simulink model "BESS_2Q_All_Cases_Pro"  (R2024b)
settings: Solver=VariableStepAuto  StartTime=0.0  StopTime=10  RelTol=1e-3
undefined symbols (not defined in the file): Down, Up
libraries: spsSeriesRLCBranchLib x30, spsIGBTDiodeLib x12, spsDCVoltageSourceLib x12, spsVoltageMeasurementLib x12, spsCurrentMeasurementLib x6, eePwmGenerator x2, slpidlib x2, spspowerguiLib x1
settings Model: Creator=jmy  LastModifiedBy=Eng.Abd-Elrhman Saad

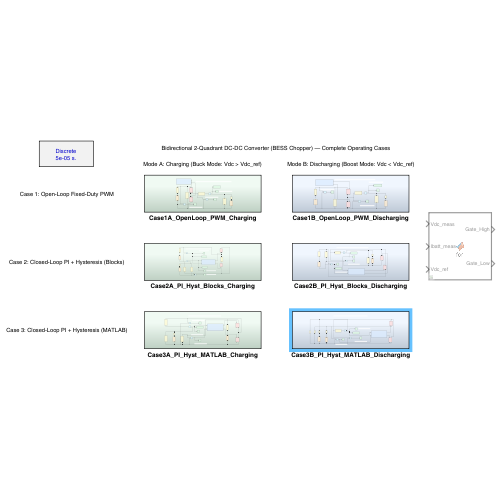
[thumbnail: Simulink's stored preview of the top-level diagram]
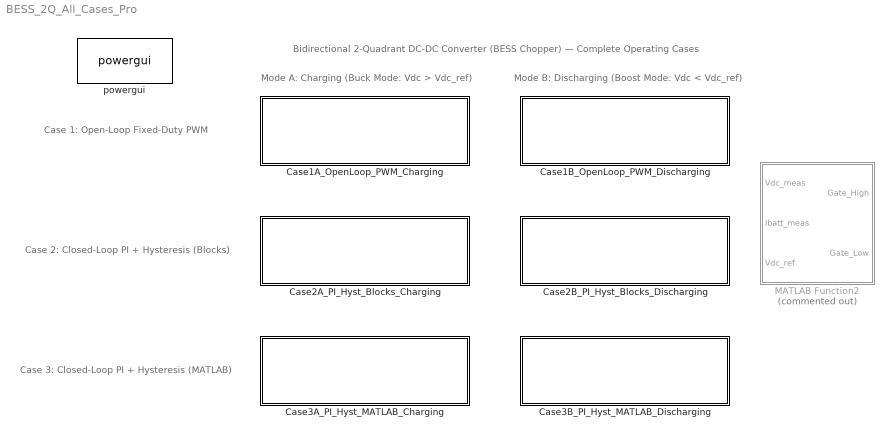
== system BESS_2Q_All_Cases_Pro ==
  note: Bidirectional 2-Quadrant DC-DC Converter (BESS Chopper) — Complete Operating Cases
  note: Mode A: Charging (Buck Mode: Vdc > Vdc_ref)
  note: Mode B: Discharging (Boost Mode: Vdc < Vdc_ref)
  note: Case 1: Open-Loop Fixed-Duty PWM
  note: Case 2: Closed-Loop PI + Hysteresis (Blocks)
  note: Case 3: Closed-Loop PI + Hysteresis (MATLAB)
  Case1A_OpenLoop_PWM_Charging : Subsystem
  Case1B_OpenLoop_PWM_Discharging : Subsystem
  Case2A_PI_Hyst_Blocks_Charging : Subsystem
  Case2B_PI_Hyst_Blocks_Discharging : Subsystem
  Case3A_PI_Hyst_MATLAB_Charging : Subsystem
  Case3B_PI_Hyst_MATLAB_Discharging : Subsystem
  MATLAB Function2 : MATLAB Function  Commented=on  TreatAsAtomicUnit=on
  powergui : spspowerguiLib/powergui  Priority=1  SimulationMode=Discrete  SampleTime=50e-6  frequency=60  Iterations=50  frequencyindice=0  Pbase=100e6  ErrMax=1e-4  UnitsV=kV  UnitsW=MW  buscounter=0  FunctionMessages=off  echomessages=off  EnableUseOfTLC=off  CurrentSourceSwitches=off  DisableSnubberDevices=off  DisableRonSwitches=off  DisableVfSwitches=off  DisplayEquations=off  AutomaticDiscreteSolvers=off  SolverType=Tustin/Backward Euler (TBE)  Interpol=off  ExternalGateDelay=off  methode=off  Ts=100  x0status=blocks  SPID=on  SwTol=0  HookPort=off  NonlinearTolerance=1e-4  nMaxIteration=100  ContinueOnMaxIteration=off  RestoreLinks=warning  ResistiveCurrentMeasurement=off  Frange=[0:2:500]  Ylog=off  Xlog=on  ShowGrid=off  save=off  variable=ZData  structure=0  ZoomFFT=off  StartTime=0.0  cycles=1  DisplayStyle=1  fundamental=60  FreqAxis=off  MaxFrequency=1000  frequencyindicesteady=1  RmsSteady=1  display=off

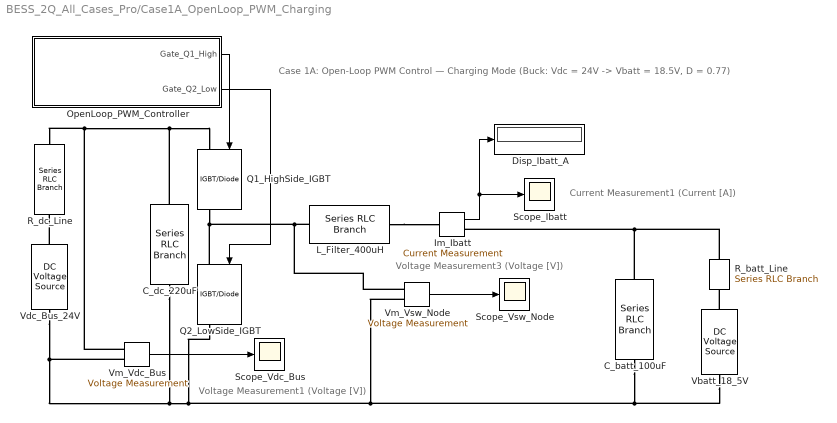
== system BESS_2Q_All_Cases_Pro/Case1A_OpenLoop_PWM_Charging ==
  note: Case 1A: Open-Loop PWM Control — Charging Mode (Buck: Vdc = 24V -> Vbatt = 18.5V, D = 0.77)
  note: Current Measurement1 (Current [A])
  note: Voltage Measurement1 (Voltage [V])
  note: Voltage Measurement3 (Voltage [V])
  C_batt_100uF : spsSeriesRLCBranchLib/Series RLC Branch  LConnTagsString=__new0  RConnTagsString=__new0  BranchType=C  Resistance=1  Inductance=400e-6  SetiL0=off  InitialCurrent=0  Capacitance=100e-6  Setx0=off  InitialVoltage=0  Measurements=None
  C_dc_220uF : spsSeriesRLCBranchLib/Series RLC Branch  LConnTagsString=__new0  RConnTagsString=__new0  BranchType=C  Resistance=1  Inductance=400e-6  SetiL0=off  InitialCurrent=0  Capacitance=220e-6  Setx0=off  InitialVoltage=0  Measurements=None
  Disp_Ibatt_A : Display
  Im_Ibatt : spsCurrentMeasurementLib/Current Measurement  PhasorSimulation=off  OutputType=Complex  PSBequivalent=0
  L_Filter_400uH : spsSeriesRLCBranchLib/Series RLC Branch  LConnTagsString=__new0  RConnTagsString=__new0  BranchType=L  Resistance=1  Inductance=400e-6  SetiL0=off  InitialCurrent=0  Capacitance=1e-6  Setx0=off  InitialVoltage=0  Measurements=None
  OpenLoop_PWM_Controller : Subsystem
  Q1_HighSide_IGBT : spsIGBTDiodeLib/IGBT//Diode  Ron=1e-3  Rs=1e5  Cs=inf  Measurements=on
  Q2_LowSide_IGBT : spsIGBTDiodeLib/IGBT//Diode  Ron=1e-3  Rs=1e5  Cs=inf  Measurements=on
  R_batt_Line : spsSeriesRLCBranchLib/Series RLC Branch  LConnTagsString=__new0  RConnTagsString=__new0  BranchType=R  Resistance=0.0001  Inductance=400e-6  SetiL0=off  InitialCurrent=0  Capacitance=220e-6  Setx0=off  InitialVoltage=0  Measurements=None
  R_dc_Line : spsSeriesRLCBranchLib/Series RLC Branch  LConnTagsString=__new0  RConnTagsString=__new0  BranchType=R  Resistance=0.0001  Inductance=400e-6  SetiL0=off  InitialCurrent=0  Capacitance=220e-6  Setx0=off  InitialVoltage=0  Measurements=None
  Scope_Ibatt : Scope
  Scope_Vdc_Bus : Scope
  Scope_Vsw_Node : Scope
  Vbatt_18_5V : spsDCVoltageSourceLib/DC Voltage Source  Amplitude=18.5  Measurements=None
  Vdc_Bus_24V : spsDCVoltageSourceLib/DC Voltage Source  Amplitude=24  Measurements=None
  Vm_Vdc_Bus : spsVoltageMeasurementLib/Voltage Measurement  PhasorSimulation=off  OutputType=Complex  PSBequivalent=0
  Vm_Vsw_Node : spsVoltageMeasurementLib/Voltage Measurement  PhasorSimulation=off  OutputType=Complex  PSBequivalent=0
  wires:
  Im_Ibatt/1 -> Disp_Ibatt_A/1, Scope_Ibatt/1
  Vm_Vsw_Node/1 -> Scope_Vsw_Node/1
  Vm_Vdc_Bus/1 -> Scope_Vdc_Bus/1
  OpenLoop_PWM_Controller/1(Gate_Q1_High) -> Q1_HighSide_IGBT/1
  OpenLoop_PWM_Controller/2(Gate_Q2_Low) -> Q2_LowSide_IGBT/1
  connections:
  Vbatt_18_5V/RConn1 -- R_batt_Line/RConn1
  Q2_LowSide_IGBT/LConn1 -- Vm_Vsw_Node/LConn1 -- L_Filter_400uH/LConn1 -- Q1_HighSide_IGBT/RConn1
  Vm_Vdc_Bus/LConn1 -- R_dc_Line/LConn1 -- C_dc_220uF/LConn1 -- Q1_HighSide_IGBT/LConn1
  R_batt_Line/LConn1 -- C_batt_100uF/LConn1 -- Im_Ibatt/RConn1
  Vm_Vdc_Bus/LConn2 -- C_dc_220uF/RConn1 -- Vbatt_18_5V/LConn1 -- C_batt_100uF/RConn1 -- Vm_Vsw_Node/LConn2 -- Q2_LowSide_IGBT/RConn1 -- Vdc_Bus_24V/LConn1
  L_Filter_400uH/RConn1 -- Im_Ibatt/LConn1
  Vdc_Bus_24V/RConn1 -- R_dc_Line/RConn1

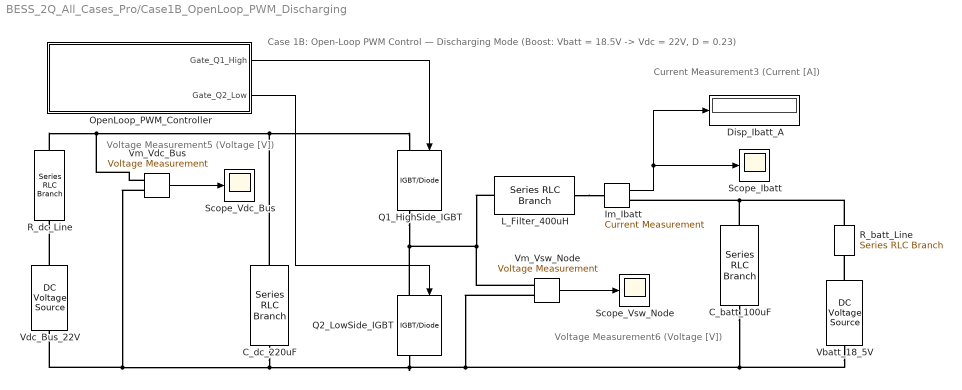
== system BESS_2Q_All_Cases_Pro/Case1B_OpenLoop_PWM_Discharging ==
  note: Case 1B: Open-Loop PWM Control — Discharging Mode (Boost: Vbatt = 18.5V -> Vdc = 22V, D = 0.23)
  note: Current Measurement3 (Current [A])
  note: Voltage Measurement5 (Voltage [V])
  note: Voltage Measurement6 (Voltage [V])
  C_batt_100uF : spsSeriesRLCBranchLib/Series RLC Branch  LConnTagsString=__new0  RConnTagsString=__new0  BranchType=C  Resistance=1  Inductance=400e-6  SetiL0=off  InitialCurrent=0  Capacitance=100e-6  Setx0=off  InitialVoltage=0  Measurements=None
  C_dc_220uF : spsSeriesRLCBranchLib/Series RLC Branch  LConnTagsString=__new0  RConnTagsString=__new0  BranchType=C  Resistance=1  Inductance=400e-6  SetiL0=off  InitialCurrent=0  Capacitance=220e-6  Setx0=off  InitialVoltage=0  Measurements=None
  Disp_Ibatt_A : Display
  Im_Ibatt : spsCurrentMeasurementLib/Current Measurement  PhasorSimulation=off  OutputType=Complex  PSBequivalent=0
  L_Filter_400uH : spsSeriesRLCBranchLib/Series RLC Branch  LConnTagsString=__new0  RConnTagsString=__new0  BranchType=L  Resistance=1  Inductance=400e-6  SetiL0=off  InitialCurrent=0  Capacitance=1e-6  Setx0=off  InitialVoltage=0  Measurements=None
  OpenLoop_PWM_Controller : Subsystem
  Q1_HighSide_IGBT : spsIGBTDiodeLib/IGBT//Diode  Ron=1e-3  Rs=1e5  Cs=inf  Measurements=on
  Q2_LowSide_IGBT : spsIGBTDiodeLib/IGBT//Diode  Ron=1e-3  Rs=1e5  Cs=inf  Measurements=on
  R_batt_Line : spsSeriesRLCBranchLib/Series RLC Branch  LConnTagsString=__new0  RConnTagsString=__new0  BranchType=R  Resistance=0.0001  Inductance=400e-6  SetiL0=off  InitialCurrent=0  Capacitance=220e-6  Setx0=off  InitialVoltage=0  Measurements=None
  R_dc_Line : spsSeriesRLCBranchLib/Series RLC Branch  LConnTagsString=__new0  RConnTagsString=__new0  BranchType=R  Resistance=0.0001  Inductance=400e-6  SetiL0=off  InitialCurrent=0  Capacitance=220e-6  Setx0=off  InitialVoltage=0  Measurements=None
  Scope_Ibatt : Scope
  Scope_Vdc_Bus : Scope
  Scope_Vsw_Node : Scope
  Vbatt_18_5V : spsDCVoltageSourceLib/DC Voltage Source  Amplitude=18.5  Measurements=None
  Vdc_Bus_22V : spsDCVoltageSourceLib/DC Voltage Source  Amplitude=22  Measurements=None
  Vm_Vdc_Bus : spsVoltageMeasurementLib/Voltage Measurement  PhasorSimulation=off  OutputType=Complex  PSBequivalent=0
  Vm_Vsw_Node : spsVoltageMeasurementLib/Voltage Measurement  PhasorSimulation=off  OutputType=Complex  PSBequivalent=0
  wires:
  Vm_Vsw_Node/1 -> Scope_Vsw_Node/1
  Im_Ibatt/1 -> Disp_Ibatt_A/1, Scope_Ibatt/1
  Vm_Vdc_Bus/1 -> Scope_Vdc_Bus/1
  OpenLoop_PWM_Controller/1(Gate_Q1_High) -> Q1_HighSide_IGBT/1
  OpenLoop_PWM_Controller/2(Gate_Q2_Low) -> Q2_LowSide_IGBT/1
  connections:
  Q1_HighSide_IGBT/LConn1 -- Vm_Vdc_Bus/LConn1 -- R_dc_Line/LConn1 -- C_dc_220uF/LConn1
  L_Filter_400uH/RConn1 -- Im_Ibatt/LConn1
  Q2_LowSide_IGBT/RConn1 -- Vdc_Bus_22V/LConn1 -- Vm_Vdc_Bus/LConn2 -- C_dc_220uF/RConn1 -- Vbatt_18_5V/LConn1 -- C_batt_100uF/RConn1 -- Vm_Vsw_Node/LConn2
  Vdc_Bus_22V/RConn1 -- R_dc_Line/RConn1
  Q2_LowSide_IGBT/LConn1 -- Q1_HighSide_IGBT/RConn1 -- L_Filter_400uH/LConn1 -- Vm_Vsw_Node/LConn1
  Vbatt_18_5V/RConn1 -- R_batt_Line/RConn1
  R_batt_Line/LConn1 -- C_batt_100uF/LConn1 -- Im_Ibatt/RConn1

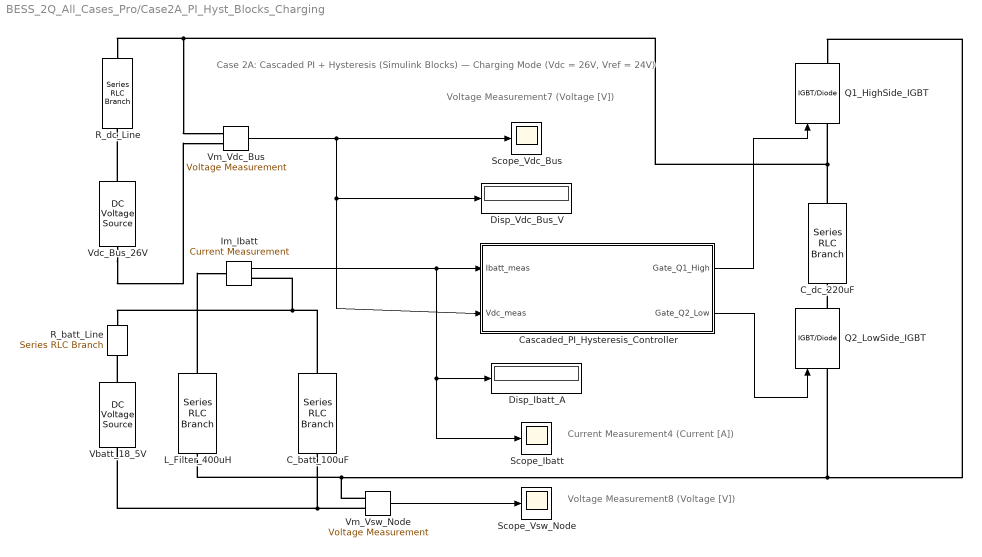
== system BESS_2Q_All_Cases_Pro/Case2A_PI_Hyst_Blocks_Charging ==
  note: Case 2A: Cascaded PI + Hysteresis (Simulink Blocks) — Charging Mode (Vdc = 26V, Vref = 24V)
  note: Current Measurement4 (Current [A])
  note: Voltage Measurement7 (Voltage [V])
  note: Voltage Measurement8 (Voltage [V])
  C_batt_100uF : spsSeriesRLCBranchLib/Series RLC Branch  LConnTagsString=__new0  RConnTagsString=__new0  BranchType=C  Resistance=1  Inductance=400e-6  SetiL0=off  InitialCurrent=0  Capacitance=100e-6  Setx0=off  InitialVoltage=0  Measurements=None
  C_dc_220uF : spsSeriesRLCBranchLib/Series RLC Branch  LConnTagsString=__new0  RConnTagsString=__new0  BranchType=C  Resistance=1  Inductance=400e-6  SetiL0=off  InitialCurrent=0  Capacitance=220e-6  Setx0=off  InitialVoltage=0  Measurements=None
  Cascaded_PI_Hysteresis_Controller : Subsystem
  Disp_Ibatt_A : Display
  Disp_Vdc_Bus_V : Display
  Im_Ibatt : spsCurrentMeasurementLib/Current Measurement  PhasorSimulation=off  OutputType=Complex  PSBequivalent=0
  L_Filter_400uH : spsSeriesRLCBranchLib/Series RLC Branch  LConnTagsString=__new0  RConnTagsString=__new0  BranchType=L  Resistance=1  Inductance=400e-6  SetiL0=off  InitialCurrent=0  Capacitance=1e-6  Setx0=off  InitialVoltage=0  Measurements=None
  Q1_HighSide_IGBT : spsIGBTDiodeLib/IGBT//Diode  Ron=1e-3  Rs=1e5  Cs=inf  Measurements=on
  Q2_LowSide_IGBT : spsIGBTDiodeLib/IGBT//Diode  Ron=1e-3  Rs=1e5  Cs=inf  Measurements=on
  R_batt_Line : spsSeriesRLCBranchLib/Series RLC Branch  LConnTagsString=__new0  RConnTagsString=__new0  BranchType=R  Resistance=0.0001  Inductance=400e-6  SetiL0=off  InitialCurrent=0  Capacitance=220e-6  Setx0=off  InitialVoltage=0  Measurements=None
  R_dc_Line : spsSeriesRLCBranchLib/Series RLC Branch  LConnTagsString=__new0  RConnTagsString=__new0  BranchType=R  Resistance=0.0001  Inductance=400e-6  SetiL0=off  InitialCurrent=0  Capacitance=220e-6  Setx0=off  InitialVoltage=0  Measurements=None
  Scope_Ibatt : Scope
  Scope_Vdc_Bus : Scope
  Scope_Vsw_Node : Scope
  Vbatt_18_5V : spsDCVoltageSourceLib/DC Voltage Source  Amplitude=18.5  Measurements=None
  Vdc_Bus_26V : spsDCVoltageSourceLib/DC Voltage Source  Amplitude=26  Measurements=None
  Vm_Vdc_Bus : spsVoltageMeasurementLib/Voltage Measurement  PhasorSimulation=off  OutputType=Complex  PSBequivalent=0
  Vm_Vsw_Node : spsVoltageMeasurementLib/Voltage Measurement  PhasorSimulation=off  OutputType=Complex  PSBequivalent=0
  wires:
  Vm_Vsw_Node/1 -> Scope_Vsw_Node/1
  Vm_Vdc_Bus/1 -> Disp_Vdc_Bus_V/1, Cascaded_PI_Hysteresis_Controller/2(Vdc_meas), Scope_Vdc_Bus/1
  Im_Ibatt/1 -> Disp_Ibatt_A/1, Scope_Ibatt/1, Cascaded_PI_Hysteresis_Controller/1(Ibatt_meas)
  Cascaded_PI_Hysteresis_Controller/1(Gate_Q1_High) -> Q1_HighSide_IGBT/1
  Cascaded_PI_Hysteresis_Controller/2(Gate_Q2_Low) -> Q2_LowSide_IGBT/1
  connections:
  Vm_Vsw_Node/LConn2 -- Vbatt_18_5V/LConn1 -- C_batt_100uF/RConn1
  Vm_Vsw_Node/LConn1 -- Q2_LowSide_IGBT/LConn1 -- Q1_HighSide_IGBT/RConn1 -- L_Filter_400uH/LConn1
  Vdc_Bus_26V/RConn1 -- R_dc_Line/RConn1
  Vdc_Bus_26V/LConn1 -- Vm_Vdc_Bus/LConn2
  L_Filter_400uH/RConn1 -- Im_Ibatt/LConn1
  Vbatt_18_5V/RConn1 -- R_batt_Line/RConn1
  C_batt_100uF/LConn1 -- Im_Ibatt/RConn1 -- R_batt_Line/LConn1
  Q2_LowSide_IGBT/RConn1 -- C_dc_220uF/RConn1
  C_dc_220uF/LConn1 -- Q1_HighSide_IGBT/LConn1 -- R_dc_Line/LConn1 -- Vm_Vdc_Bus/LConn1

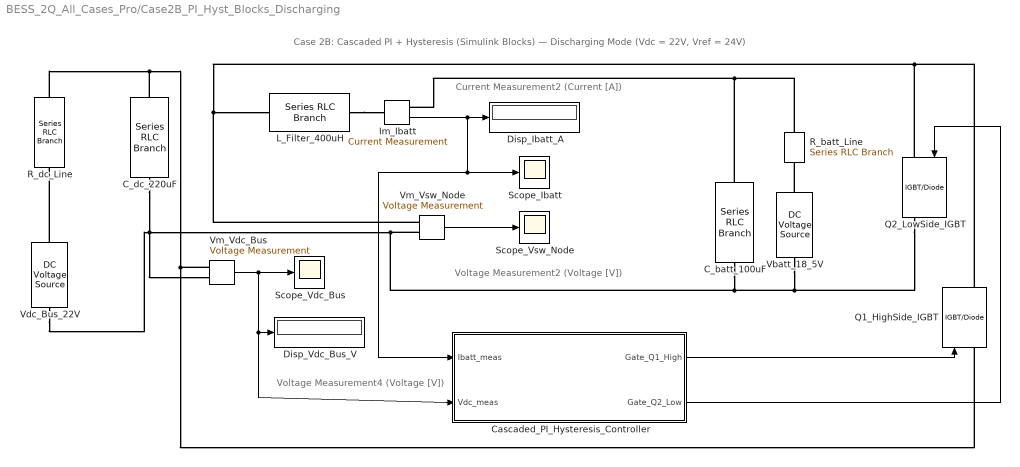
== system BESS_2Q_All_Cases_Pro/Case2B_PI_Hyst_Blocks_Discharging ==
  note: Case 2B: Cascaded PI + Hysteresis (Simulink Blocks) — Discharging Mode (Vdc = 22V, Vref = 24V)
  note: Current Measurement2 (Current [A])
  note: Voltage Measurement2 (Voltage [V])
  note: Voltage Measurement4 (Voltage [V])
  C_batt_100uF : spsSeriesRLCBranchLib/Series RLC Branch  LConnTagsString=__new0  RConnTagsString=__new0  BranchType=C  Resistance=1  Inductance=400e-6  SetiL0=off  InitialCurrent=0  Capacitance=100e-6  Setx0=off  InitialVoltage=0  Measurements=None
  C_dc_220uF : spsSeriesRLCBranchLib/Series RLC Branch  LConnTagsString=__new0  RConnTagsString=__new0  BranchType=C  Resistance=1  Inductance=400e-6  SetiL0=off  InitialCurrent=0  Capacitance=220e-6  Setx0=off  InitialVoltage=0  Measurements=None
  Cascaded_PI_Hysteresis_Controller : Subsystem
  Disp_Ibatt_A : Display
  Disp_Vdc_Bus_V : Display
  Im_Ibatt : spsCurrentMeasurementLib/Current Measurement  PhasorSimulation=off  OutputType=Complex  PSBequivalent=0
  L_Filter_400uH : spsSeriesRLCBranchLib/Series RLC Branch  LConnTagsString=__new0  RConnTagsString=__new0  BranchType=L  Resistance=1  Inductance=400e-6  SetiL0=off  InitialCurrent=0  Capacitance=1e-6  Setx0=off  InitialVoltage=0  Measurements=None
  Q1_HighSide_IGBT : spsIGBTDiodeLib/IGBT//Diode  Ron=1e-3  Rs=1e5  Cs=inf  Measurements=on
  Q2_LowSide_IGBT : spsIGBTDiodeLib/IGBT//Diode  Ron=1e-3  Rs=1e5  Cs=inf  Measurements=on
  R_batt_Line : spsSeriesRLCBranchLib/Series RLC Branch  LConnTagsString=__new0  RConnTagsString=__new0  BranchType=R  Resistance=0.0001  Inductance=400e-6  SetiL0=off  InitialCurrent=0  Capacitance=220e-6  Setx0=off  InitialVoltage=0  Measurements=None
  R_dc_Line : spsSeriesRLCBranchLib/Series RLC Branch  LConnTagsString=__new0  RConnTagsString=__new0  BranchType=R  Resistance=0.0001  Inductance=400e-6  SetiL0=off  InitialCurrent=0  Capacitance=220e-6  Setx0=off  InitialVoltage=0  Measurements=None
  Scope_Ibatt : Scope
  Scope_Vdc_Bus : Scope
  Scope_Vsw_Node : Scope
  Vbatt_18_5V : spsDCVoltageSourceLib/DC Voltage Source  Amplitude=18.5  Measurements=None
  Vdc_Bus_22V : spsDCVoltageSourceLib/DC Voltage Source  Amplitude=22  Measurements=None
  Vm_Vdc_Bus : spsVoltageMeasurementLib/Voltage Measurement  PhasorSimulation=off  OutputType=Complex  PSBequivalent=0
  Vm_Vsw_Node : spsVoltageMeasurementLib/Voltage Measurement  PhasorSimulation=off  OutputType=Complex  PSBequivalent=0
  wires:
  Vm_Vdc_Bus/1 -> Cascaded_PI_Hysteresis_Controller/2(Vdc_meas), Disp_Vdc_Bus_V/1, Scope_Vdc_Bus/1
  Im_Ibatt/1 -> Disp_Ibatt_A/1, Scope_Ibatt/1, Cascaded_PI_Hysteresis_Controller/1(Ibatt_meas)
  Vm_Vsw_Node/1 -> Scope_Vsw_Node/1
  Cascaded_PI_Hysteresis_Controller/1(Gate_Q1_High) -> Q1_HighSide_IGBT/1
  Cascaded_PI_Hysteresis_Controller/2(Gate_Q2_Low) -> Q2_LowSide_IGBT/1
  connections:
  Vdc_Bus_22V/RConn1 -- R_dc_Line/RConn1
  Q2_LowSide_IGBT/RConn1 -- Vbatt_18_5V/LConn1 -- C_batt_100uF/RConn1 -- Vdc_Bus_22V/LConn1 -- Vm_Vdc_Bus/LConn2 -- C_dc_220uF/RConn1 -- Vm_Vsw_Node/LConn2
  Vbatt_18_5V/RConn1 -- R_batt_Line/RConn1
  R_batt_Line/LConn1 -- C_batt_100uF/LConn1 -- Im_Ibatt/RConn1
  Q2_LowSide_IGBT/LConn1 -- Q1_HighSide_IGBT/RConn1 -- Vm_Vsw_Node/LConn1 -- L_Filter_400uH/LConn1
  R_dc_Line/LConn1 -- Q1_HighSide_IGBT/LConn1 -- Vm_Vdc_Bus/LConn1 -- C_dc_220uF/LConn1
  L_Filter_400uH/RConn1 -- Im_Ibatt/LConn1

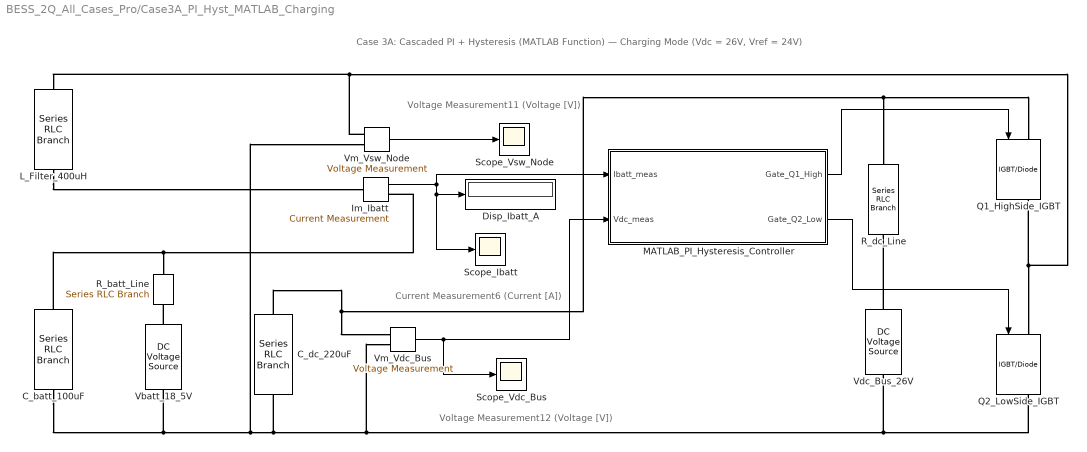
== system BESS_2Q_All_Cases_Pro/Case3A_PI_Hyst_MATLAB_Charging ==
  note: Case 3A: Cascaded PI + Hysteresis (MATLAB Function) — Charging Mode (Vdc = 26V, Vref = 24V)
  note: Current Measurement6 (Current [A])
  note: Voltage Measurement12 (Voltage [V])
  note: Voltage Measurement11 (Voltage [V])
  C_batt_100uF : spsSeriesRLCBranchLib/Series RLC Branch  LConnTagsString=__new0  RConnTagsString=__new0  BranchType=C  Resistance=1  Inductance=400e-6  SetiL0=off  InitialCurrent=0  Capacitance=100e-6  Setx0=off  InitialVoltage=0  Measurements=None
  C_dc_220uF : spsSeriesRLCBranchLib/Series RLC Branch  LConnTagsString=__new0  RConnTagsString=__new0  BranchType=C  Resistance=1  Inductance=400e-6  SetiL0=off  InitialCurrent=0  Capacitance=220e-6  Setx0=off  InitialVoltage=0  Measurements=None
  Disp_Ibatt_A : Display
  Im_Ibatt : spsCurrentMeasurementLib/Current Measurement  PhasorSimulation=off  OutputType=Complex  PSBequivalent=0
  L_Filter_400uH : spsSeriesRLCBranchLib/Series RLC Branch  LConnTagsString=__new0  RConnTagsString=__new0  BranchType=L  Resistance=1  Inductance=400e-6  SetiL0=off  InitialCurrent=0  Capacitance=1e-6  Setx0=off  InitialVoltage=0  Measurements=None
  MATLAB_PI_Hysteresis_Controller : Subsystem
  Q1_HighSide_IGBT : spsIGBTDiodeLib/IGBT//Diode  Ron=1e-3  Rs=1e5  Cs=inf  Measurements=on
  Q2_LowSide_IGBT : spsIGBTDiodeLib/IGBT//Diode  Ron=1e-3  Rs=1e5  Cs=inf  Measurements=on
  R_batt_Line : spsSeriesRLCBranchLib/Series RLC Branch  LConnTagsString=__new0  RConnTagsString=__new0  BranchType=R  Resistance=0.0001  Inductance=400e-6  SetiL0=off  InitialCurrent=0  Capacitance=220e-6  Setx0=off  InitialVoltage=0  Measurements=None
  R_dc_Line : spsSeriesRLCBranchLib/Series RLC Branch  LConnTagsString=__new0  RConnTagsString=__new0  BranchType=R  Resistance=0.0001  Inductance=400e-6  SetiL0=off  InitialCurrent=0  Capacitance=220e-6  Setx0=off  InitialVoltage=0  Measurements=None
  Scope_Ibatt : Scope
  Scope_Vdc_Bus : Scope
  Scope_Vsw_Node : Scope
  Vbatt_18_5V : spsDCVoltageSourceLib/DC Voltage Source  Amplitude=18.5  Measurements=None
  Vdc_Bus_26V : spsDCVoltageSourceLib/DC Voltage Source  Amplitude=26  Measurements=None
  Vm_Vdc_Bus : spsVoltageMeasurementLib/Voltage Measurement  PhasorSimulation=off  OutputType=Complex  PSBequivalent=0
  Vm_Vsw_Node : spsVoltageMeasurementLib/Voltage Measurement  PhasorSimulation=off  OutputType=Complex  PSBequivalent=0
  wires:
  Vm_Vsw_Node/1 -> Scope_Vsw_Node/1
  Vm_Vdc_Bus/1 -> MATLAB_PI_Hysteresis_Controller/2(Vdc_meas), Scope_Vdc_Bus/1
  Im_Ibatt/1 -> Scope_Ibatt/1, Disp_Ibatt_A/1, MATLAB_PI_Hysteresis_Controller/1(Ibatt_meas)
  MATLAB_PI_Hysteresis_Controller/1(Gate_Q1_High) -> Q1_HighSide_IGBT/1
  MATLAB_PI_Hysteresis_Controller/2(Gate_Q2_Low) -> Q2_LowSide_IGBT/1
  connections:
  Vdc_Bus_26V/RConn1 -- R_dc_Line/RConn1
  C_batt_100uF/RConn1 -- Vbatt_18_5V/LConn1 -- C_dc_220uF/RConn1 -- Vm_Vdc_Bus/LConn2 -- Vdc_Bus_26V/LConn1 -- Q2_LowSide_IGBT/RConn1 -- Vm_Vsw_Node/LConn2
  C_batt_100uF/LConn1 -- R_batt_Line/LConn1 -- Im_Ibatt/RConn1
  Vm_Vsw_Node/LConn1 -- L_Filter_400uH/LConn1 -- Q2_LowSide_IGBT/LConn1 -- Q1_HighSide_IGBT/RConn1
  C_dc_220uF/LConn1 -- R_dc_Line/LConn1 -- Q1_HighSide_IGBT/LConn1 -- Vm_Vdc_Bus/LConn1
  Vbatt_18_5V/RConn1 -- R_batt_Line/RConn1
  L_Filter_400uH/RConn1 -- Im_Ibatt/LConn1

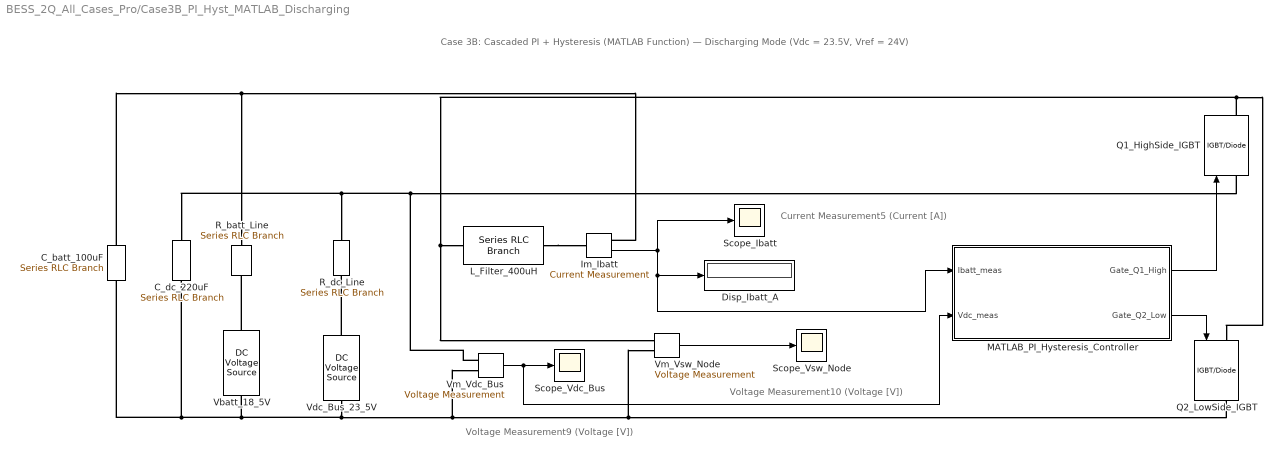
== system BESS_2Q_All_Cases_Pro/Case3B_PI_Hyst_MATLAB_Discharging ==
  note: Case 3B: Cascaded PI + Hysteresis (MATLAB Function) — Discharging Mode (Vdc = 23.5V, Vref = 24V)
  note: Current Measurement5 (Current [A])
  note: Voltage Measurement9 (Voltage [V])
  note: Voltage Measurement10 (Voltage [V])
  C_batt_100uF : spsSeriesRLCBranchLib/Series RLC Branch  LConnTagsString=__new0  RConnTagsString=__new0  BranchType=C  Resistance=1  Inductance=400e-6  SetiL0=off  InitialCurrent=0  Capacitance=100e-6  Setx0=off  InitialVoltage=0  Measurements=None
  C_dc_220uF : spsSeriesRLCBranchLib/Series RLC Branch  LConnTagsString=__new0  RConnTagsString=__new0  BranchType=C  Resistance=1  Inductance=400e-6  SetiL0=off  InitialCurrent=0  Capacitance=220e-6  Setx0=off  InitialVoltage=0  Measurements=None
  Disp_Ibatt_A : Display
  Im_Ibatt : spsCurrentMeasurementLib/Current Measurement  PhasorSimulation=off  OutputType=Complex  PSBequivalent=0
  L_Filter_400uH : spsSeriesRLCBranchLib/Series RLC Branch  LConnTagsString=__new0  RConnTagsString=__new0  BranchType=L  Resistance=1  Inductance=400e-6  SetiL0=off  InitialCurrent=0  Capacitance=1e-6  Setx0=off  InitialVoltage=0  Measurements=None
  MATLAB_PI_Hysteresis_Controller : Subsystem
  Q1_HighSide_IGBT : spsIGBTDiodeLib/IGBT//Diode  Ron=1e-3  Rs=1e5  Cs=inf  Measurements=on
  Q2_LowSide_IGBT : spsIGBTDiodeLib/IGBT//Diode  Ron=1e-3  Rs=1e5  Cs=inf  Measurements=on
  R_batt_Line : spsSeriesRLCBranchLib/Series RLC Branch  LConnTagsString=__new0  RConnTagsString=__new0  BranchType=R  Resistance=0.0001  Inductance=400e-6  SetiL0=off  InitialCurrent=0  Capacitance=220e-6  Setx0=off  InitialVoltage=0  Measurements=None
  R_dc_Line : spsSeriesRLCBranchLib/Series RLC Branch  LConnTagsString=__new0  RConnTagsString=__new0  BranchType=R  Resistance=0.0001  Inductance=400e-6  SetiL0=off  InitialCurrent=0  Capacitance=220e-6  Setx0=off  InitialVoltage=0  Measurements=None
  Scope_Ibatt : Scope
  Scope_Vdc_Bus : Scope
  Scope_Vsw_Node : Scope
  Vbatt_18_5V : spsDCVoltageSourceLib/DC Voltage Source  Amplitude=18.5  Measurements=None
  Vdc_Bus_23_5V : spsDCVoltageSourceLib/DC Voltage Source  Amplitude=23.5  Measurements=None
  Vm_Vdc_Bus : spsVoltageMeasurementLib/Voltage Measurement  PhasorSimulation=off  OutputType=Complex  PSBequivalent=0
  Vm_Vsw_Node : spsVoltageMeasurementLib/Voltage Measurement  PhasorSimulation=off  OutputType=Complex  PSBequivalent=0
  wires:
  Vm_Vdc_Bus/1 -> MATLAB_PI_Hysteresis_Controller/2(Vdc_meas), Scope_Vdc_Bus/1
  Vm_Vsw_Node/1 -> Scope_Vsw_Node/1
  Im_Ibatt/1 -> MATLAB_PI_Hysteresis_Controller/1(Ibatt_meas), Disp_Ibatt_A/1, Scope_Ibatt/1
  MATLAB_PI_Hysteresis_Controller/1(Gate_Q1_High) -> Q1_HighSide_IGBT/1
  MATLAB_PI_Hysteresis_Controller/2(Gate_Q2_Low) -> Q2_LowSide_IGBT/1
  connections:
  Vdc_Bus_23_5V/LConn1 -- C_batt_100uF/RConn1 -- C_dc_220uF/RConn1 -- Vbatt_18_5V/LConn1 -- Vm_Vdc_Bus/LConn2 -- Q2_LowSide_IGBT/RConn1 -- Vm_Vsw_Node/LConn2
  Vdc_Bus_23_5V/RConn1 -- R_dc_Line/RConn1
  Q1_HighSide_IGBT/RConn1 -- Q2_LowSide_IGBT/LConn1 -- L_Filter_400uH/LConn1 -- Vm_Vsw_Node/LConn1
  Vm_Vdc_Bus/LConn1 -- R_dc_Line/LConn1 -- C_dc_220uF/LConn1 -- Q1_HighSide_IGBT/LConn1
  C_batt_100uF/LConn1 -- Im_Ibatt/RConn1 -- R_batt_Line/LConn1
  Vbatt_18_5V/RConn1 -- R_batt_Line/RConn1
  L_Filter_400uH/RConn1 -- Im_Ibatt/LConn1

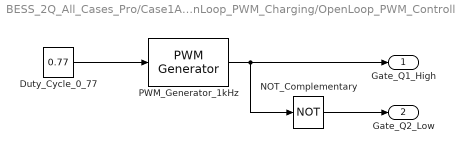
== system BESS_2Q_All_Cases_Pro/Case1A_OpenLoop_PWM_Charging/OpenLoop_PWM_Controller ==
  Duty_Cycle_0_77 : Constant  Value=0.77
  NOT_Complementary : Logic  Operator=NOT  IconShape=distinctive  AllPortsSameDT=off  OutDataTypeStr=boolean
  PWM_Generator_1kHz : eePwmGenerator/PWM Generator  CarrCount=Up-Down  Tper=0.001  Tdelay=0  Ts=5e-5
  Gate_Q1_High : Outport
  Gate_Q2_Low : Outport  Port=2
  wires:
  PWM_Generator_1kHz/1 -> Gate_Q1_High/1, NOT_Complementary/1
  NOT_Complementary/1 -> Gate_Q2_Low/1
  Duty_Cycle_0_77/1 -> PWM_Generator_1kHz/1

== system BESS_2Q_All_Cases_Pro/Case1B_OpenLoop_PWM_Discharging/OpenLoop_PWM_Controller ==
  Duty_Cycle_0_23 : Constant  Value=0.23
  NOT_Complementary : Logic  Operator=NOT  IconShape=distinctive  AllPortsSameDT=off  OutDataTypeStr=boolean
  PWM_Generator_1kHz : eePwmGenerator/PWM Generator  CarrCount=Up-Down  Tper=0.001  Tdelay=0  Ts=5e-5
  Gate_Q1_High : Outport
  Gate_Q2_Low : Outport  Port=2
  wires:
  PWM_Generator_1kHz/1 -> NOT_Complementary/1, Gate_Q2_Low/1
  Duty_Cycle_0_23/1 -> PWM_Generator_1kHz/1
  NOT_Complementary/1 -> Gate_Q1_High/1

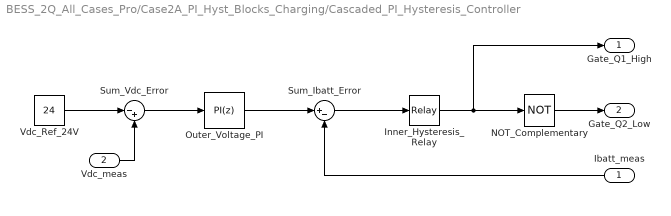
== system BESS_2Q_All_Cases_Pro/Case2A_PI_Hyst_Blocks_Charging/Cascaded_PI_Hysteresis_Controller ==
  Ibatt_meas : Inport
  Vdc_meas : Inport  Port=2
  Inner_Hysteresis_Relay : Relay  OnSwitchValue=0.5  OffSwitchValue=-0.5
  NOT_Complementary : Logic  Operator=NOT  IconShape=distinctive  AllPortsSameDT=off  OutDataTypeStr=boolean
  Outer_Voltage_PI : slpidlib/PID Controller  Controller=PI  Form=Parallel  TimeDomain=Discrete-time  UseExternalTs=off  SampleTime=-1  IntegratorMethod=Forward Euler  FilterMethod=Forward Euler  ControllerParametersSource=internal  P=0.1  I=10  UseKiTs=off  D=0  UseExternalDerivativeSource=off  N=100  UseFilter=on  TunerSelectOption=Transfer Function Based (PID Tuner App)  InitialConditionSource=internal  InitialConditionForIntegrator=0  InitialConditionForFilter=0  DifferentiatorICPrevScaledInput=0  ExternalReset=none  TrackingMode=off  Kt=1  LimitOutput=on  SatLimitsSource=internal  UpperSaturationLimit=3.1  LowerSaturationLimit=-10  LinearizeAsGain=off  AntiWindupMode=none  Kb=1  LimitIntegrator=off  UpperIntegratorSaturationLimit=inf  LowerIntegratorSaturationLimit=-inf  POutMin=[]  POutMax=[]  IOutMin=[]  IOutMax=[]  DOutMin=[]  DOutMax=[]  NOutMin=[]  NOutMax=[]  SumOutMin=[]  SumOutMax=[]  SaturationOutMin=[]  SaturationOutMax=[]  PParamMin=[]  PParamMax=[]  IParamMin=[]  IParamMax=[]  DParamMin=[]  DParamMax=[]  NParamMin=[]  NParamMax=[]  KbParamMin=[]  KbParamMax=[]  KtParamMin=[]  KtParamMax=[]  KbOutMin=[]  KbOutMax=[]  KtOutMin=[]  KtOutMax=[]  IntegratorOutMin=[]  IntegratorOutMax=[]  FilterOutMin=[]  FilterOutMax=[]  SumI1OutMin=[]  SumI1OutMax=[]  SumI2OutMin=[]  SumI2OutMax=[]  SumI3OutMin=[]  SumI3OutMax=[]  SumI4OutMin=[]  SumI4OutMax=[]  SumDOutMin=[]  SumDOutMax=[]  DifferentiatorOutMin=[]  DifferentiatorOutMax=[]  FilterDiffOutCoefMin=[]  FilterDiffOutCoefMax=[]  ReciprocalOutMin=[]  ReciprocalOutMax=[]  SumDenOutMin=[]  SumDenOutMax=[]  SumNumOutMin=[]  SumNumOutMax=[]  DivideOutMin=[]  DivideOutMax=[]  UdiffTsProdOutMin=[]  UdiffTsProdOutMax=[]  NTsProdOutMin=[]  NTsProdOutMax=[]  UintegralTsProdOutMin=[]  UintegralTsProdOutMax=[]  UngainTsProdOutMin=[]  UngainTsProdOutMax=[]  ClampingZeroOutDataTypeStr=Inherit: Inherit via back propagation  ClampingZeroOutMin=[]  ClampingZeroOutMax=[]  FilterDenConstantOutDataTypeStr=Inherit: Inherit via back propagation  FilterDenConstantOutMin=[]  FilterDenConstantOutMax=[]  PCopyOutDataTypeStr=Inherit: Inherit via back propagation  PCopyOutMin=[]  PCopyOutMax=[]  NCopyOutDataTypeStr=Inherit: Inherit via back propagation  NCopyOutMin=[]  NCopyOutMax=[]  IntegratorContinuousStateAttributes=''  IntegratorStateMustResolveToSignalObject=off  IntegratorRTWStateStorageClass=Auto  FilterContinuousStateAttributes=''  FilterStateMustResolveToSignalObject=off  FilterRTWStateStorageClass=Auto  ParallelPVariant=InternalParameters  IdealPVariant=Disabled  IVariant=InternalParameters  DVariant=Disabled  IntegratorVariant=Discrete  SatVariant=Enabled  AWVariant=Passthrough  PCopyVariant=Disabled  TRVariant=Disabled  FdbkBlocksVariant=Forward  IdealPFdbkVariant=Disabled  SatFdbkVariant=Disabled  DerivativeFilterVariant=Disabled  NVariant=Disabled  NCopyVariant=Disabled_SignalSpec  FilterICVariant=Disabled  IntegratorICVariant=InternalICs  ExternalResetVariant=Disabled  TRSumVariant=Passthrough  SumFdbkVariant=Disabled  SumVariant=Sum_PI  TsampFilterVariant=InternalTs  TsampNgainVariant=Passthrough  TsampIntegralVariant=Disabled_SignalSpec  ExternalSaturationOutDataTypeStr=Inherit: Same as second input  DerivativeSourceVariant=Disabled  PreIntVariant=InternalPreInt
  Sum_Ibatt_Error : Sum  Inputs=|+-
  Sum_Vdc_Error : Sum  Inputs=|-+
  Vdc_Ref_24V : Constant  Value=24
  Gate_Q1_High : Outport
  Gate_Q2_Low : Outport  Port=2
  wires:
  Inner_Hysteresis_Relay/1 -> Gate_Q1_High/1, NOT_Complementary/1
  Sum_Vdc_Error/1 -> Outer_Voltage_PI/1
  Outer_Voltage_PI/1 -> Sum_Ibatt_Error/1
  Sum_Ibatt_Error/1 -> Inner_Hysteresis_Relay/1
  NOT_Complementary/1 -> Gate_Q2_Low/1
  Vdc_meas/1 -> Sum_Vdc_Error/2
  Vdc_Ref_24V/1 -> Sum_Vdc_Error/1
  Ibatt_meas/1 -> Sum_Ibatt_Error/2

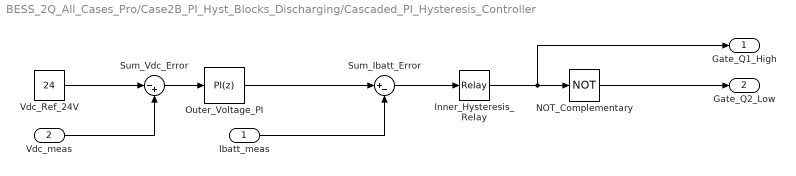
== system BESS_2Q_All_Cases_Pro/Case2B_PI_Hyst_Blocks_Discharging/Cascaded_PI_Hysteresis_Controller ==
  Ibatt_meas : Inport
  Vdc_meas : Inport  Port=2
  Inner_Hysteresis_Relay : Relay  OnSwitchValue=0.5  OffSwitchValue=-0.5
  NOT_Complementary : Logic  Operator=NOT  IconShape=distinctive  AllPortsSameDT=off  OutDataTypeStr=boolean
  Outer_Voltage_PI : slpidlib/PID Controller  Controller=PI  Form=Parallel  TimeDomain=Discrete-time  UseExternalTs=off  SampleTime=-1  IntegratorMethod=Forward Euler  FilterMethod=Forward Euler  ControllerParametersSource=internal  P=0.1  I=10  UseKiTs=off  D=0  UseExternalDerivativeSource=off  N=100  UseFilter=on  TunerSelectOption=Transfer Function Based (PID Tuner App)  InitialConditionSource=internal  InitialConditionForIntegrator=0  InitialConditionForFilter=0  DifferentiatorICPrevScaledInput=0  ExternalReset=none  TrackingMode=off  Kt=1  LimitOutput=on  SatLimitsSource=internal  UpperSaturationLimit=3.1  LowerSaturationLimit=-10  LinearizeAsGain=off  AntiWindupMode=none  Kb=1  LimitIntegrator=off  UpperIntegratorSaturationLimit=inf  LowerIntegratorSaturationLimit=-inf  POutMin=[]  POutMax=[]  IOutMin=[]  IOutMax=[]  DOutMin=[]  DOutMax=[]  NOutMin=[]  NOutMax=[]  SumOutMin=[]  SumOutMax=[]  SaturationOutMin=[]  SaturationOutMax=[]  PParamMin=[]  PParamMax=[]  IParamMin=[]  IParamMax=[]  DParamMin=[]  DParamMax=[]  NParamMin=[]  NParamMax=[]  KbParamMin=[]  KbParamMax=[]  KtParamMin=[]  KtParamMax=[]  KbOutMin=[]  KbOutMax=[]  KtOutMin=[]  KtOutMax=[]  IntegratorOutMin=[]  IntegratorOutMax=[]  FilterOutMin=[]  FilterOutMax=[]  SumI1OutMin=[]  SumI1OutMax=[]  SumI2OutMin=[]  SumI2OutMax=[]  SumI3OutMin=[]  SumI3OutMax=[]  SumI4OutMin=[]  SumI4OutMax=[]  SumDOutMin=[]  SumDOutMax=[]  DifferentiatorOutMin=[]  DifferentiatorOutMax=[]  FilterDiffOutCoefMin=[]  FilterDiffOutCoefMax=[]  ReciprocalOutMin=[]  ReciprocalOutMax=[]  SumDenOutMin=[]  SumDenOutMax=[]  SumNumOutMin=[]  SumNumOutMax=[]  DivideOutMin=[]  DivideOutMax=[]  UdiffTsProdOutMin=[]  UdiffTsProdOutMax=[]  NTsProdOutMin=[]  NTsProdOutMax=[]  UintegralTsProdOutMin=[]  UintegralTsProdOutMax=[]  UngainTsProdOutMin=[]  UngainTsProdOutMax=[]  ClampingZeroOutDataTypeStr=Inherit: Inherit via back propagation  ClampingZeroOutMin=[]  ClampingZeroOutMax=[]  FilterDenConstantOutDataTypeStr=Inherit: Inherit via back propagation  FilterDenConstantOutMin=[]  FilterDenConstantOutMax=[]  PCopyOutDataTypeStr=Inherit: Inherit via back propagation  PCopyOutMin=[]  PCopyOutMax=[]  NCopyOutDataTypeStr=Inherit: Inherit via back propagation  NCopyOutMin=[]  NCopyOutMax=[]  IntegratorContinuousStateAttributes=''  IntegratorStateMustResolveToSignalObject=off  IntegratorRTWStateStorageClass=Auto  FilterContinuousStateAttributes=''  FilterStateMustResolveToSignalObject=off  FilterRTWStateStorageClass=Auto  ParallelPVariant=InternalParameters  IdealPVariant=Disabled  IVariant=InternalParameters  DVariant=Disabled  IntegratorVariant=Discrete  SatVariant=Enabled  AWVariant=Passthrough  PCopyVariant=Disabled  TRVariant=Disabled  FdbkBlocksVariant=Forward  IdealPFdbkVariant=Disabled  SatFdbkVariant=Disabled  DerivativeFilterVariant=Disabled  NVariant=Disabled  NCopyVariant=Disabled_SignalSpec  FilterICVariant=Disabled  IntegratorICVariant=InternalICs  ExternalResetVariant=Disabled  TRSumVariant=Passthrough  SumFdbkVariant=Disabled  SumVariant=Sum_PI  TsampFilterVariant=InternalTs  TsampNgainVariant=Passthrough  TsampIntegralVariant=Disabled_SignalSpec  ExternalSaturationOutDataTypeStr=Inherit: Same as second input  DerivativeSourceVariant=Disabled  PreIntVariant=InternalPreInt
  Sum_Ibatt_Error : Sum  Inputs=|+-
  Sum_Vdc_Error : Sum  Inputs=|-+
  Vdc_Ref_24V : Constant  Value=24
  Gate_Q1_High : Outport
  Gate_Q2_Low : Outport  Port=2
  wires:
  Sum_Ibatt_Error/1 -> Inner_Hysteresis_Relay/1
  Vdc_meas/1 -> Sum_Vdc_Error/2
  Vdc_Ref_24V/1 -> Sum_Vdc_Error/1
  Outer_Voltage_PI/1 -> Sum_Ibatt_Error/1
  Sum_Vdc_Error/1 -> Outer_Voltage_PI/1
  Inner_Hysteresis_Relay/1 -> NOT_Complementary/1, Gate_Q1_High/1
  Ibatt_meas/1 -> Sum_Ibatt_Error/2
  NOT_Complementary/1 -> Gate_Q2_Low/1

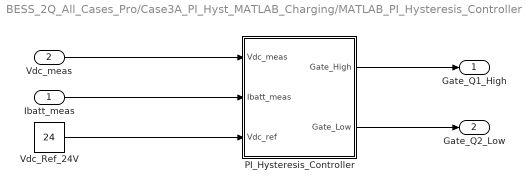
== system BESS_2Q_All_Cases_Pro/Case3A_PI_Hyst_MATLAB_Charging/MATLAB_PI_Hysteresis_Controller ==
  Ibatt_meas : Inport
  Vdc_meas : Inport  Port=2
  PI_Hysteresis_Controller : MATLAB Function  TreatAsAtomicUnit=on
  Vdc_Ref_24V : Constant  Value=24
  Gate_Q1_High : Outport
  Gate_Q2_Low : Outport  Port=2
  wires:
  Vdc_Ref_24V/1 -> PI_Hysteresis_Controller/3(Vdc_ref)
  Vdc_meas/1 -> PI_Hysteresis_Controller/1(Vdc_meas)
  PI_Hysteresis_Controller/2(Gate_Low) -> Gate_Q2_Low/1
  PI_Hysteresis_Controller/1(Gate_High) -> Gate_Q1_High/1
  Ibatt_meas/1 -> PI_Hysteresis_Controller/2(Ibatt_meas)

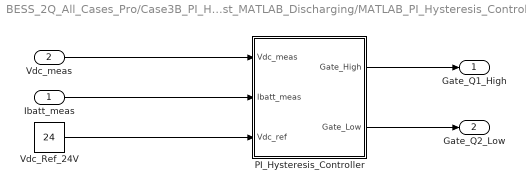
== system BESS_2Q_All_Cases_Pro/Case3B_PI_Hyst_MATLAB_Discharging/MATLAB_PI_Hysteresis_Controller ==
  Ibatt_meas : Inport
  Vdc_meas : Inport  Port=2
  PI_Hysteresis_Controller : MATLAB Function  TreatAsAtomicUnit=on
  Vdc_Ref_24V : Constant  Value=24
  Gate_Q1_High : Outport
  Gate_Q2_Low : Outport  Port=2
  wires:
  Vdc_meas/1 -> PI_Hysteresis_Controller/1(Vdc_meas)
  Vdc_Ref_24V/1 -> PI_Hysteresis_Controller/3(Vdc_ref)
  Ibatt_meas/1 -> PI_Hysteresis_Controller/2(Ibatt_meas)
  PI_Hysteresis_Controller/2(Gate_Low) -> Gate_Q2_Low/1
  PI_Hysteresis_Controller/1(Gate_High) -> Gate_Q1_High/1

== matlab function BESS_2Q_All_Cases_Pro/Case3A_PI_Hyst_MATLAB_Charging/MATLAB_PI_Hysteresis_Controller/PI_Hysteresis_Controller ==
  data: Vdc_meas input; Gate_High output; Ibatt_meas input; Vdc_ref input; Gate_Low output
function [Gate_High, Gate_Low] = fcn(Vdc_meas, Ibatt_meas, Vdc_ref)
    % --- PART 1: Memory (Persistent Variables) ---
    persistent int_err_v S_high
    if isempty(int_err_v)
        int_err_v = 0;
        S_high = 0;
    end

    % --- Internal Constants ---
    Ts = 5e-5;      % Sampling time (from your powergui)
    h = 0.01;        % Hysteresis band
    Kp_v = 0.1;     % PI Proportional Gain
    Ki_v = 10;      % PI Integral Gain

    % --- PART 2: Outer Loop (Voltage PI Control) ---
    err_v = Vdc_meas - Vdc_ref ;
    int_err_v = int_err_v + err_v * Ts;
    
    % Anti-windup (Clamping the integrator)
    int_err_v = max(min(int_err_v, 5), -5); 
    
    % Calculate the Current Reference (I_ref)
    I_ref = (Kp_v * err_v) + (Ki_v * int_err_v);

    % --- PART 3: Current Saturation (Protection) ---
    % Logic: Charging = Positive (+3.1A max), Discharging = Negative (-10A max)
    I_max_charge = 3.1;   
    I_max_disch  = -10.0; 
    
    % This line is Part 3: It clamps the reference to your hardware limits
    I_ref_sat = max(I_max_disch, min(I_max_charge, I_ref));

    % --- PART 4: Inner Loop (Hysteresis Current Control) ---
    % S_high = 1: Top IGBT ON (Increases current)
    % S_high = 0: Bottom IGBT ON (Decreases current)
    if Ibatt_meas < (I_ref_sat - h)
        S_high = 1;
    elseif Ibatt_meas > (I_ref_sat + h)
        S_high = 0;
    end

    % --- PART 5: Gate Outputs ---
    Gate_High = S_high;
    Gate_Low  = 1 - S_high; % Complementary switching
end

== matlab function BESS_2Q_All_Cases_Pro/Case3B_PI_Hyst_MATLAB_Discharging/MATLAB_PI_Hysteresis_Controller/PI_Hysteresis_Controller ==
  data: Vdc_meas input; Gate_High output; Ibatt_meas input; Vdc_ref input; Gate_Low output
function [Gate_High, Gate_Low] = fcn(Vdc_meas, Ibatt_meas, Vdc_ref)
    % --- PART 1: Memory (Persistent Variables) ---
    persistent int_err_v S_high
    if isempty(int_err_v)
        int_err_v = 0;
        S_high = 0;
    end

    % --- Internal Constants ---
    Ts = 5e-5;      % Sampling time (from your powergui)
    h = 0.05;        % Hysteresis band
    Kp_v = 0.1;     % PI Proportional Gain
    Ki_v = 10;      % PI Integral Gain

    % --- PART 2: Outer Loop (Voltage PI Control) ---
    err_v = Vdc_meas - Vdc_ref ;
    int_err_v = int_err_v + err_v * Ts;
    
    % Anti-windup (Clamping the integrator)
    int_err_v = max(min(int_err_v, 5), -5); 
    
    % Calculate the Current Reference (I_ref)
    I_ref = (Kp_v * err_v) + (Ki_v * int_err_v);

    % --- PART 3: Current Saturation (Protection) ---
    % Logic: Charging = Positive (+3.1A max), Discharging = Negative (-10A max)
    I_max_charge = 3.1;   
    I_max_disch  = -10.0; 
    
    % This line is Part 3: It clamps the reference to your hardware limits
    I_ref_sat = max(I_max_disch, min(I_max_charge, I_ref));

    % --- PART 4: Inner Loop (Hysteresis Current Control) ---
    % S_high = 1: Top IGBT ON (Increases current)
    % S_high = 0: Bottom IGBT ON (Decreases current)
    if Ibatt_meas < (I_ref_sat - h)
        S_high = 1;
    elseif Ibatt_meas > (I_ref_sat + h)
        S_high = 0;
    end

    % --- PART 5: Gate Outputs ---
    Gate_High = S_high;
    Gate_Low  = 1 - S_high; % Complementary switching
end

== matlab function BESS_2Q_All_Cases_Pro/MATLAB Function2 ==
  data: Vdc_meas input; Gate_High output; Ibatt_meas input; Vdc_ref input; Gate_Low output
function [Gate_High, Gate_Low] = fcn(Vdc_meas, Ibatt_meas, Vdc_ref)
    % Persistent variables for the PI integrator and switch state
    persistent int_err_v S_high
    if isempty(int_err_v)
        int_err_v = 0;
        S_high = 0;
    end

    % --- Internal Constants ---
    Ts = 5e-5;            % Matches your PowerGUI (50 microseconds)
    h = 0.1;              % Hysteresis band (Fixed at 0.1 Amperes)
    
    % PI Gains
    Kp_v = 1.2;           
    Ki_v = 35;            
    
    % Battery Safety Limits
    % Max charge: 3.1A (Negative) | Max discharge: 10A (Positive)
    I_max_disch = 10.0;
    I_max_charge = -3.1;

    % --- 1. Outer Loop: Voltage PI Control ---
    err_v = Vdc_ref - Vdc_meas;
    
    % Update integrator with anti-windup clamping
    int_err_v = int_err_v + err_v * Ts;
    int_err_v = max(min(int_err_v, 5), -5); 
    
    % Calculate desired current (I_ref)
    I_ref = (Kp_v * err_v) + (Ki_v * int_err_v);

    % Force I_ref to stay within battery specs
    if I_ref > I_max_disch
        I_ref = I_max_disch;
    elseif I_ref < I_max_charge
        I_ref = I_max_charge;
    end

    % --- 2. Inner Loop: Hysteresis Logic ---
    % S_high = 1 -> Top IGBT closed (Increases inductor current)
    % S_high = 0 -> Bottom IGBT closed (Decreases inductor current)
    if Ibatt_meas < (I_ref - h)
        S_high = 1;
    elseif Ibatt_meas > (I_ref + h)
        S_high = 0;
    end

    % --- 3. Final Gate Outputs ---
    Gate_High = S_high;
    Gate_Low  = 1 - S_high; % Complementary signal
endfunction [Gate_High, Gate_Low] = fcn(Vdc_meas, Ibatt_meas, Vdc_ref)
